simulink model "TFT_Cluster_Model"  (R2025a)
settings: Solver=VariableStepAuto  StartTime=0.0  StopTime=10.0  RelTol=1e-3
libraries: simulink x1
settings Model: DataDictionary=TFT_Cluster_Model.sldd  Creator=nikul  LastModifiedBy=nikul

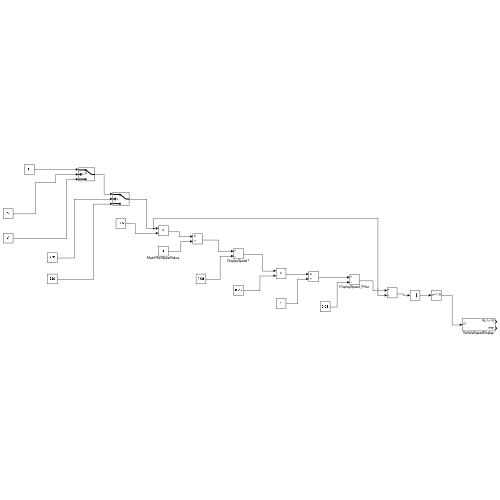
[thumbnail: Simulink's stored preview of the top-level diagram]
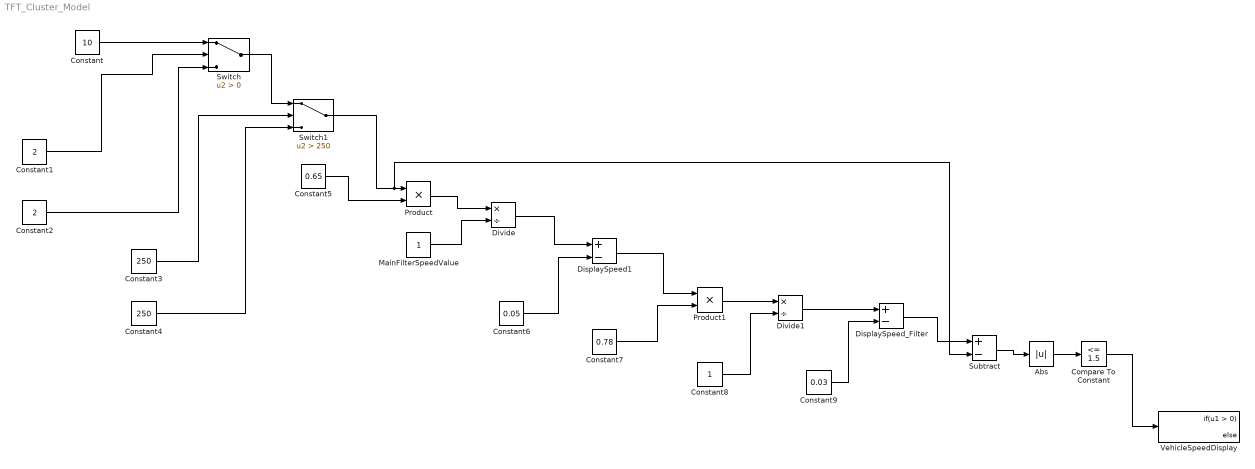
== system TFT_Cluster_Model ==
  Abs : Abs  SaturateOnIntegerOverflow=off
  Compare To Constant : simulink/Logic and Bit Operations/Compare To Constant  relop=<=  const=1.5  OutDataTypeStr=boolean
  Constant : Constant  Value=10
  Constant1 : Constant  Value=2
  Constant2 : Constant  Value=2
  Constant3 : Constant  Value=250
  Constant4 : Constant  Value=250
  Constant5 : Constant  Value=0.65
  Constant6 : Constant  Value=0.05
  Constant7 : Constant  Value=0.78
  Constant8 : Constant
  Constant9 : Constant  Value=0.03
  DisplaySpeed1 : Sum  Inputs=+-
  DisplaySpeed_Filter : Sum  Inputs=+-
  Divide : Product  Inputs=*/
  Divide1 : Product  Inputs=*/
  MainFilterSpeedValue : Constant
  Product : Product
  Product1 : Product
  Subtract : Sum  Inputs=+-
  Switch : Switch  Criteria=u2 > Threshold  SaturateOnIntegerOverflow=off  InputSameDT=off
  Switch1 : Switch  Criteria=u2 > Threshold  Threshold=250  SaturateOnIntegerOverflow=off  InputSameDT=off
  VehicleSpeedDisplay : If
  wires:
  Constant/1 -> Switch/1
  Constant1/1 -> Switch/2
  Constant2/1 -> Switch/3
  Constant3/1 -> Switch1/2
  Constant4/1 -> Switch1/3
  Switch/1 -> Switch1/1
  Switch1/1 -> Subtract/2, Product/1
  Constant5/1 -> Product/2
  Product/1 -> Divide/1
  MainFilterSpeedValue/1 -> Divide/2
  Divide/1 -> DisplaySpeed1/1
  Constant6/1 -> DisplaySpeed1/2
  DisplaySpeed1/1 -> Product1/1
  Constant7/1 -> Product1/2
  Product1/1 -> Divide1/1
  Constant8/1 -> Divide1/2
  Divide1/1 -> DisplaySpeed_Filter/1
  Constant9/1 -> DisplaySpeed_Filter/2
  DisplaySpeed_Filter/1 -> Subtract/1
  Subtract/1 -> Abs/1
  Abs/1 -> Compare To Constant/1
  Compare To Constant/1 -> VehicleSpeedDisplay/1
